simulink model "model_new_plant"  (R2024b)
settings: Solver=VariableStepAuto  StartTime=0.0  StopTime=100  RelTol=1e-3
undefined symbols (not defined in the file): K1, K2
settings Model: Creator=njpan  LastModifiedBy=jacksonwright

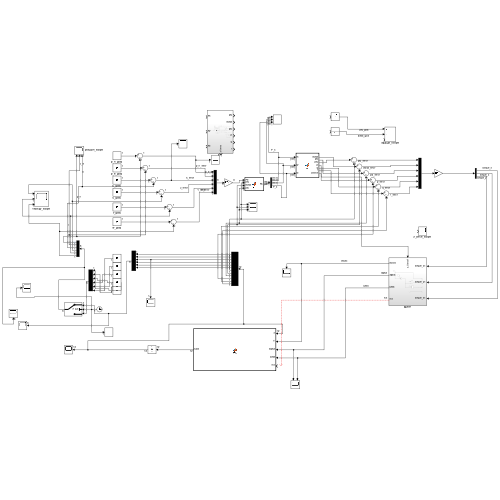
[thumbnail: Simulink's stored preview of the top-level diagram]
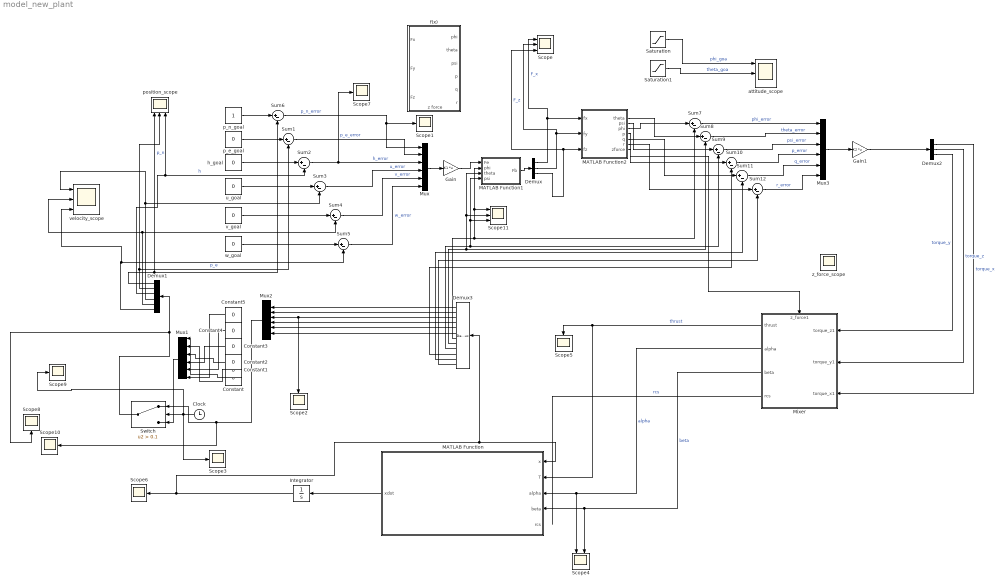
== system model_new_plant ==
  Clock : Clock
  Constant{,1..5} (6 alike) : Constant  Value=0
  Demux : Demux  Outputs=3
  Demux1 : Demux  Outputs=6
  Demux2 : Demux  Outputs=3
  Demux3 : Demux  Outputs=12
  Gain : Gain  Gain=K1  Multiplication=Matrix(K*u)
  Gain1 : Gain  Gain=K2  Multiplication=Matrix(K*u)
  Integrator : Integrator
  MATLAB Function : MATLAB Function  TreatAsAtomicUnit=on
  MATLAB Function1 : MATLAB Function  TreatAsAtomicUnit=on
  MATLAB Function2 : MATLAB Function  TreatAsAtomicUnit=on
  Mixer : Subsystem
      settings: PortSchema="{\"entries\":[{\"content\":{\"sides\":[{\"content\":{\"connectorIds\":[\"In1\",\"In2\",\"In3\"]},\"type\":\"ConnectorPlacement.EquallySpacedRectSide\",\"uuid\":\"e4ab6201-3171-425b-b678-f5a82ca77998\"},{\"content\":{\"connectorIds\":[\"Out1\",\"Out2\",\"Out3\",\"Out4\"],\"side\":\"RIGHT\"},\"type\":\"ConnectorPlacement.EquallySpacedRectSide\",\"uuid\":\"c6aae40c-8090-4a79-98d3-b60c0d3e66c5\"},{\"content\":{\"connectorIds\":[\"In4\"],\"side\":\"TOP\"},\"type\":\"ConnectorPlacement.EquallySpacedRectSide\",\"uuid\":\"89717ce5-f3d0-4b2e-8505-89723edf9773\"}]},\"type\":\"ConnectorPlacement.EquallySpacedConnector\",\"uuid\":\"ace876b5-bd23-4119-b1c7-2a296fd8fc0f\"}],\"packageUris\":[\"http://schema.mathworks.com/mf0/Connector/R2020b\"],\"version\":\"1.0\"}"
  Mux{,1..3} (4 alike) : Mux  Inputs=6
  Saturation : Saturate  UpperLimit=5*pi/180  LowerLimit=-5*pi/180
  Saturation1 : Saturate  UpperLimit=5*pi/180  LowerLimit=-5*pi/180
  Scope : Scope  NumInputPorts=3
  Scope{1..3,5..10} (9 alike) : Scope
  Scope11 : Scope  NumInputPorts=3
  Scope4 : Scope  NumInputPorts=2
  Sum{1..12} (12 alike) : Sum  Inputs=|+-
  Switch : Switch  Criteria=u2 > Threshold  Threshold=0.1  SaturateOnIntegerOverflow=off  InputSameDT=off
  attitude_scope : Scope  NumInputPorts=3
  f(x) : Subsystem
      settings: PortSchema="{\"entries\":[{\"content\":{\"sides\":[{\"content\":{\"connectorIds\":[\"In1\",\"In2\",\"In3\"]},\"type\":\"ConnectorPlacement.EquallySpacedRectSide\",\"uuid\":\"e7aeffbb-634f-4153-9868-9d3e2e4280ad\"},{\"content\":{\"connectorIds\":[\"Out1\",\"Out2\",\"Out3\",\"Out4\",\"Out5\",\"Out6\"],\"side\":\"RIGHT\"},\"type\":\"ConnectorPlacement.EquallySpacedRectSide\",\"uuid\":\"e6d97028-2a10-4268-a5e2-55bbdc39a0c5\"},{\"content\":{\"side\":\"TOP\"},\"type\":\"ConnectorPlacement.EquallySpacedRectSide\",\"uuid\":\"fa716bc0-4a18-4661-a72d-62488d70bdc1\"},{\"content\":{\"connectorIds\":[\"Out7\"],\"side\":\"BOTTOM\"},\"type\":\"ConnectorPlacement.EquallySpacedRectSide\",\"uuid\":\"f442cf4b-5896-4629-a7d3-01e27d8da1cb\"}]},\"type\":\"ConnectorPlacement.EquallySpacedConnector\",\"uuid\":\"0a376c34-a895-4dfb-85c3-cafa4de2d877\"}],\"packageUris\":[\"http://schema.mathworks.com/mf0/Connector/R2020b\"],\"version\":\"1.0\"}"
  h_goal : Constant  Value=0
  p_e_goal : Constant  Value=0
  p_n_goal : Constant
  position_scope : Scope  NumInputPorts=3
  u_goal : Constant  Value=0
  v_goal : Constant  Value=0
  velocity_scope : Scope  NumInputPorts=3
  w_goal : Constant  Value=0
  z_force_scope : Scope
  wires:
  Sum6/1 -> Mux/1, Scope1/1  "p_n_error"
  Sum1/1 -> Mux/2  "p_e_error"
  Sum2/1 -> Mux/3, Scope7/1  "h_error"
  Sum3/1 -> Mux/4  "u_error"
  Sum4/1 -> Mux/5  "v_error"
  Sum5/1 -> Mux/6  "w_error"
  h_goal/1 -> Sum2/1
  u_goal/1 -> Sum3/1
  v_goal/1 -> Sum4/1
  w_goal/1 -> Sum5/1
  Demux/3 -> Scope/3, MATLAB Function2/3(fz)  "F_z"
  p_n_goal/1 -> Sum6/1
  Sum7/1 -> Mux3/1  "phi_error"
  Sum8/1 -> Mux3/2  "theta_error"
  Sum9/1 -> Mux3/3  "psi_error"
  Sum10/1 -> Mux3/4  "p_error"
  Sum11/1 -> Mux3/5  "q_error"
  Sum12/1 -> Mux3/6  "r_error"
  Demux2/1 -> Mixer/3(torque_x1)  "torque_x"
  Demux2/3 -> Mixer/1(torque_z1)  "torque_y"
  Demux2/2 -> Mixer/2(torque_y1)  "torque_z"
  Mixer/4(rcs) -> ?  "rcs"
  Mixer/3(beta) -> MATLAB Function/4(beta), Scope4/2  "beta"
  Mixer/2(alpha) -> MATLAB Function/3(alpha), Scope4/1  "alpha"
  Mixer/1(thrust) -> Scope5/1, MATLAB Function/2(T)  "thrust"
  Demux/1 -> Scope/1, MATLAB Function2/1(fx)  "F_x"
  Gain/1 -> MATLAB Function1/1(Fe)
  Mux/1 -> Gain/1
  Clock/1 -> Scope9/1, Scope3/1, Switch/2
  Constant/1 -> Mux1/1
  Constant1/1 -> Mux1/2
  Constant2/1 -> Mux1/3
  Constant3/1 -> Mux1/4
  Constant4/1 -> Mux1/5
  Constant5/1 -> Mux1/6
  Mux1/1 -> Switch/3
  Switch/1 -> Scope8/1, Demux1/1
  Mux2/1 -> Switch/1, Scope10/1
  Demux1/1 -> position_scope/1, Sum6/2  "p_n"
  Demux1/2 -> position_scope/2, Sum1/2  "p_e"
  Demux1/3 -> position_scope/3, Sum2/2  "h"
  Demux1/4 -> velocity_scope/1, Sum3/2
  Demux1/5 -> Sum4/2, velocity_scope/2
  Demux1/6 -> velocity_scope/3, Sum5/2
  Mux3/1 -> Gain1/1
  Gain1/1 -> Demux2/1
  MATLAB Function/1(xdot) -> Integrator/1
  Integrator/1 -> MATLAB Function/1(x), Demux3/1, Scope6/1
  Demux3/12 -> Sum12/2
  Demux3/11 -> Sum11/2
  Demux3/10 -> Sum10/2
  Demux3/9 -> Sum9/2, MATLAB Function1/4(psi), Scope11/3
  Demux3/8 -> Sum8/2, Scope11/2, MATLAB Function1/3(theta)
  Demux3/7 -> MATLAB Function1/2(phi), Scope11/1, Sum7/2
  Demux3/1 -> Mux2/1
  Demux3/2 -> Mux2/2
  Demux3/3 -> Mux2/3, Scope2/1
  Demux3/4 -> Mux2/4
  Demux3/5 -> Mux2/5
  Demux3/6 -> Mux2/6
  Demux/2 -> Scope/2, MATLAB Function2/2(fy)
  p_e_goal/1 -> Sum1/1
  Saturation/1 -> attitude_scope/1  "phi_goa"
  Saturation1/1 -> attitude_scope/2  "theta_goa"
  MATLAB Function1/1(Fb) -> Demux/1
  MATLAB Function2/3(phi) -> Sum7/1
  MATLAB Function2/1(theta) -> Sum8/1
  MATLAB Function2/2(psi) -> Sum9/1
  MATLAB Function2/5(q) -> Sum11/1
  MATLAB Function2/6(r) -> Sum12/1
  MATLAB Function2/4(p) -> Sum10/1
  MATLAB Function2/7(zforce) -> Mixer/4(z_force1)

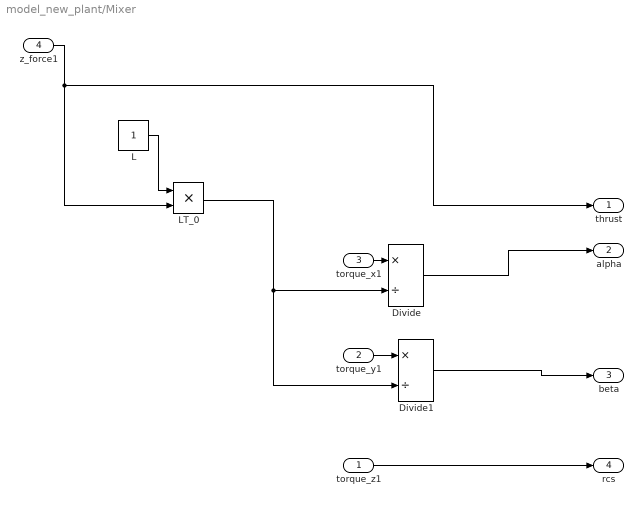
== system model_new_plant/Mixer ==
  torque_z1 : Inport
  torque_y1 : Inport  Port=2
  torque_x1 : Inport  Port=3
  z_force1 : Inport  Port=4
  Divide : Product  Inputs=*/
  Divide1 : Product  Inputs=*/
  L : Constant
  LT_0 : Product
  thrust : Outport
  alpha : Outport  Port=2
  beta : Outport  Port=3
  rcs : Outport  Port=4
  wires:
  torque_y1/1 -> Divide1/1
  Divide/1 -> alpha/1
  L/1 -> LT_0/1
  LT_0/1 -> Divide1/2, Divide/2
  torque_z1/1 -> rcs/1
  z_force1/1 -> LT_0/2, thrust/1
  Divide1/1 -> beta/1
  torque_x1/1 -> Divide/1

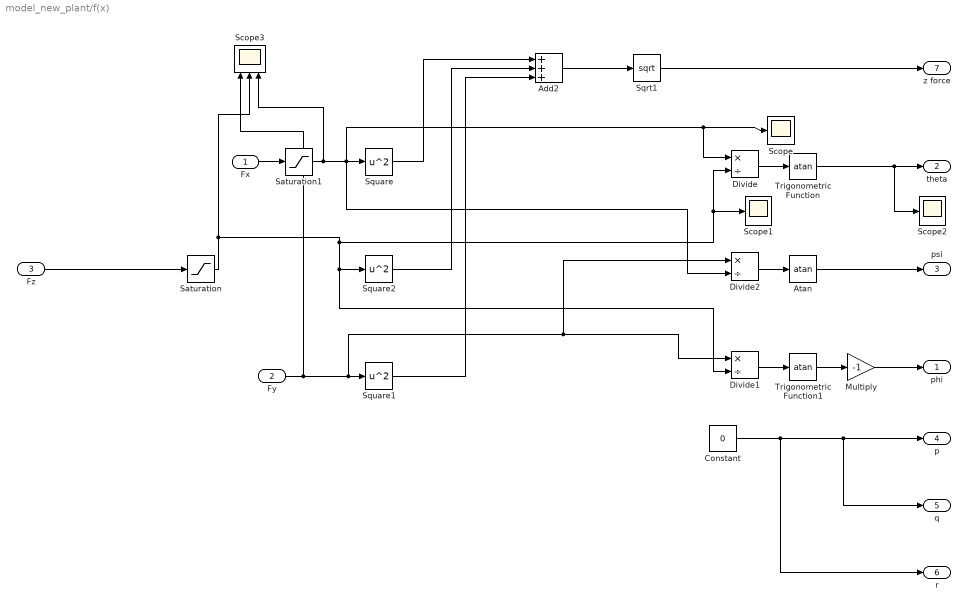
== system model_new_plant/f(x) ==
  Fx : Inport
  Fy : Inport  Port=2
  Fz : Inport  Port=3
  Add2 : Sum  Inputs=+++
  Atan : Trigonometry  Operator=atan
  Constant : Constant  Value=0
  Divide : Product  Inputs=*/
  Divide1 : Product  Inputs=*/
  Divide2 : Product  Inputs=*/
  Multiply : Gain  Gain=-1
  Saturation : Saturate  UpperLimit=Inf  LowerLimit=0.00001
  Saturation1 : Saturate  UpperLimit=Inf  LowerLimit=0.00001
  Scope : Scope
  Scope1 : Scope
  Scope2 : Scope
  Scope3 : Scope  NumInputPorts=3
  Sqrt1 : Sqrt
  Square : Math  Operator=square
  Square1 : Math  Operator=square
  Square2 : Math  Operator=square
  Trigonometric Function : Trigonometry  Operator=atan
  Trigonometric Function1 : Trigonometry  Operator=atan
  phi : Outport
  theta : Outport  Port=2
  psi : Outport  Port=3
  p : Outport  Port=4
  q : Outport  Port=5
  r : Outport  Port=6
  z force : Outport  Port=7
  wires:
  Multiply/1 -> phi/1
  Divide/1 -> Trigonometric Function/1
  Square1/1 -> Add2/3
  Square/1 -> Add2/1
  Divide1/1 -> Trigonometric Function1/1
  Atan/1 -> psi/1
  Add2/1 -> Sqrt1/1
  Square2/1 -> Add2/2
  Fy/1 -> Divide2/1, Divide1/1, Square1/1, Scope3/1
  Divide2/1 -> Atan/1
  Trigonometric Function/1 -> Scope2/1, theta/1
  Sqrt1/1 -> z force/1
  Constant/1 -> r/1, q/1, p/1
  Trigonometric Function1/1 -> Multiply/1
  Saturation/1 -> Scope3/2, Divide/2, Scope1/1, Square2/1, Divide1/2
  Fz/1 -> Saturation/1
  Fx/1 -> Saturation1/1
  Saturation1/1 -> Divide2/2, Divide/1, Scope/1, Square/1, Scope3/3

== matlab function model_new_plant/MATLAB Function1 ==
  data: Fe input; Fb output; phi input; theta input; psi input
function Fb = fcn(Fe, phi,theta,psi)

Rx = [1, 0, 0;
    0, cos(phi), -sin(phi);
    0, sin(phi), cos(phi)]

Ry = [cos(theta), 0, sin(theta);
    0, 1, 0;
    -sin(theta), 0, cos(theta)]

Rz = [cos(psi), sin(psi), 0;
    sin(psi), cos(psi), 0;
    0, 0, 1]

rotMat = Rz*Ry*Rx

Fe(3) = Fe(3) + 9.81


Fb = rotMat*Fe;

== matlab function model_new_plant/MATLAB Function ==
  data: x input; T input; xdot output size=12; alpha input; beta input; rcs input
 function xdot = fcn(x, T, alpha, beta, rcs)

xdot = [0 0 0 0 0 0 0 0 0 0 0 0]';

m = 1;
g = 9.81;
L = 1;
Ixx = 5;
Iyy = 5;
Izz = 5;

% pn = x(1);
% pe = x(2);
% pu = x(3);
u = x(4);
v = x(5);
w = x(6);
phi = x(7);
theta = x(8);
psi = x(9);
p = x(10);
q = x(11);
r = x(12);

xdot(2) = cos(theta)*cos(psi)*u + (sin(phi)*sin(theta)*cos(psi) - cos(phi)*sin(psi))*v + (cos(phi)*sin(theta)*cos(psi)+sin(phi)*sin(psi))*w;
xdot(1) = cos(theta)*sin(psi)*u + (sin(phi)*sin(theta)*sin(psi)+cos(phi)*cos(psi))*v + (cos(phi)*sin(theta)*sin(psi)-sin(phi)*cos(psi))*w;
xdot(3) = (sin(theta)*u - sin(phi)*cos(theta)*v + cos(phi)*cos(theta)*w);
xdot(4) = r*v - q*w + (T*sin(alpha)*cos(beta) + m*g*sin(theta))/m;
xdot(5) = p*w - r*u + (T*sin(beta)*cos(alpha) - m*g*cos(theta)*sin(phi))/m;
xdot(6) = q*u - p*v + (T*cos(alpha)*cos(beta) - m*g*cos(theta)*cos(phi))/m;
xdot(7) = p + sin(phi)*tan(theta)*q + cos(phi)*tan(theta)*r;
xdot(8) = cos(phi)*q - sin(phi)*r;
xdot(9) = sin(phi)/cos(theta)*q + cos(phi)/cos(theta)*r;
xdot(10) = (Iyy - Izz)*q*r/Ixx + L*T*sin(alpha)/Ixx;
xdot(11) = (Izz - Ixx)*p*r/Ixx - L*T*sin(beta)/Iyy;
xdot(12) = (Ixx - Iyy)*p*q/Izz + rcs/Izz;
end

== matlab function model_new_plant/MATLAB Function2 ==
  data: fx input; theta output; fy input; fz input; psi output; phi output; p output; q output; r output; zforce output
function [theta,psi,phi,p,q,r,zforce]= fcn(fx,fy,fz)

% zforce
zforce = sqrt(((fx)^2)+((fy)^2)+((fz)^2));

% angular velocities are zero
p = 0;
q = 0;
r = 0;

% angle goals
% as we near our goal, the angle gets smaller

% psi/yaw
if (fx > 10) 
    phi = 10 * (pi/180);
elseif (fx > 5)
    phi = 5 * (pi/180);
elseif (fx > 1)
    phi = 3 * (pi/180);
elseif (1 > fx > 0)
    phi = 1 * (pi/180);
else 
    phi = 0; 
end

% phi/roll
if fy > 10
    theta = 10 * (pi/180);
elseif fz > 5
    theta = 5 * (pi/180);
elseif fz > 1
    theta = 3 * (pi/180);
elseif (1 > fz > 0)
    theta = 1 * (pi/180);
else
    theta = 0; 
end

psi = 0


% theta/pitch
% if fz == 0
%     theta = 0; % this was we can account for when fz = 0
% else
%     theta = atan(fx / fz);
% end
function y = fcn(u)

y = u;
